simulink model "SIMULINKADVANCED"  (R2026a)
settings: Solver=VariableStepAuto  StopTime=0.08
undefined symbols (not defined in the file or in its folder): k_FF
libraries: cstblocks_lti x4
settings Model: Creator=raffaellamoccia  LastModifiedBy=raffaellamoccia

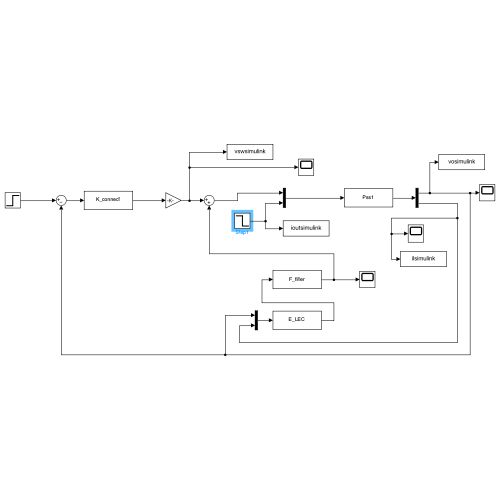
[thumbnail: Simulink's stored preview of the top-level diagram]
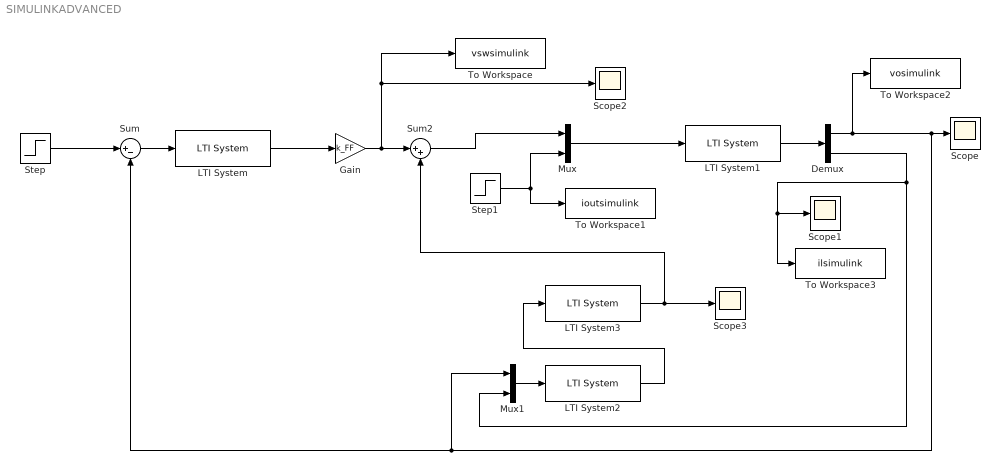
== system SIMULINKADVANCED ==
  Demux : Demux  Outputs=2
  Gain : Gain  Gain=k_FF
  LTI System : cstblocks_lti/LTI System  sys=K_connect  IC=[]  PadeOrder=0
      settings: LibrarySourceBlock=cstblocks/LTI System
  LTI System1 : cstblocks_lti/LTI System  sys=Pss1  IC=[]  PadeOrder=0
      settings: LibrarySourceBlock=cstblocks/LTI System
  LTI System2 : cstblocks_lti/LTI System  sys=E_LEC  IC=[]  PadeOrder=0
      settings: LibrarySourceBlock=cstblocks/LTI System
  LTI System3 : cstblocks_lti/LTI System  sys=F_filter  IC=[]  PadeOrder=0
      settings: LibrarySourceBlock=cstblocks/LTI System
  Mux : Mux  Inputs=2
  Mux1 : Mux  Inputs=2
  Scope{,1..3} (4 alike) : Scope
      Scope settings: ActiveDisplayYMinimum=4.9996515214117041  ActiveDisplayYMaximum=5.0005546953313731
      Scope1 settings: MaximizeAxes=On  ShowGrid=off  ActiveDisplayYMinimum=265.07210352058109  ActiveDisplayYMaximum=389.13123161498743
      Scope2 settings: ActiveDisplayYMinimum=5.0335585301358039  ActiveDisplayYMaximum=5.0432703488319319  DataLoggingVariableName=ScopeData2
      Scope3 settings: ActiveDisplayYMinimum=-0.0034534199873444476  ActiveDisplayYMaximum=-0.00075640810298492384  DataLoggingVariableName=ScopeData3
  Step : Step  Time=0  FinalValue=5  SampleTime=0
  Step1 : Step  Time=0.005  FinalValue=-0.5  SampleTime=0
  Sum : Sum  Inputs=|+-
  Sum2 : Sum  Inputs=|++
  To Workspace : ToWorkspace  VariableName=vswsimulink  SaveFormat=Timeseries  SampleTime=-1
  To Workspace1 : ToWorkspace  VariableName=ioutsimulink  SaveFormat=Timeseries  SampleTime=-1
  To Workspace2 : ToWorkspace  VariableName=vosimulink  SaveFormat=Timeseries  SampleTime=-1
  To Workspace3 : ToWorkspace  VariableName=ilsimulink  SaveFormat=Timeseries  SampleTime=-1
  wires:
  LTI System1/1 -> Demux/1
  Sum/1 -> LTI System/1
  Gain/1 -> Scope2/1, To Workspace/1, Sum2/1
  Step/1 -> Sum/1
  Step1/1 -> To Workspace1/1, Mux/2
  Mux/1 -> LTI System1/1
  Demux/1 -> To Workspace2/1, Scope/1, Sum/2, Mux1/1
  Demux/2 -> Scope1/1, To Workspace3/1, Mux1/2
  LTI System/1 -> Gain/1
  Mux1/1 -> LTI System2/1
  LTI System2/1 -> LTI System3/1
  LTI System3/1 -> Scope3/1, Sum2/2
  Sum2/1 -> Mux/1
